simulink model "AttitudeControl_Sim"  (R2017b)
settings: Solver=ode4  StartTime=0.0  StopTime=10  FixedStep=0.001  RelTol=1e-3
InitFcn:
  | if exist('Init_control.m','file')
  | Init_control;
  | end
values from neighbouring files (symbols this model uses):
  DEG2RAD = 0.0174533    [Init_control.m]
  Kd_YAW_AngleRate = 0.00    (= 0)    [Init_control.m]
  Ki_YAW_AngleRate = 0.01    [Init_control.m]
  Kp_YAW_AngleRate = 0.5    [Init_control.m]
  MAX_CONTROL_ANGLE_PITCH = 35    [Init_control.m]
  MAX_CONTROL_ANGLE_RATE_PITCH = 220    [Init_control.m]
  MAX_CONTROL_ANGLE_RATE_ROLL = 220    [Init_control.m]
  MAX_CONTROL_ANGLE_RATE_Y = 200    [Init_control.m]
  MAX_CONTROL_ANGLE_ROLL = 35    [Init_control.m]
  ModelInit_AngEuler = [0, 0, 0]    [Init.m]    (also in Init_control.m)
  ModelInit_PosE = [0, 0, 0]    [Init.m]    (also in Init_control.m)
  ModelInit_Rads = 0    [Init.m]    (also in Init_control.m)
  ModelInit_RateB = [0, 0, 0]    [Init.m]    (also in Init_control.m)
  ModelInit_VelB = [0, 0, 0]    [Init.m]    (also in Init_control.m)
  ModelParam_envGravityAcc = 9.8    [Init.m]
  ModelParam_motorCr = 1148    [Init.m]
  ModelParam_motorJm = 0.0001287    [Init.m]
  ModelParam_motorT = 0.02    [Init.m]
  ModelParam_motorWb = -141.4    [Init.m]
  ModelParam_rotorCm = 1.779e-07    [Init.m]
  ModelParam_rotorCt = 1.105e-05    [Init.m]
  ModelParam_uavCCm = [0.0035 0.0039 0.0034]    [Init.m]
  ModelParam_uavCd = 0.055    [Init.m]
  ModelParam_uavJ = [ModelParam_uavJxx, 0, 0;     0, ModelParam_uavJyy, 0;     0, 0, ModelParam_uavJzz]    [Init.m]
  ModelParam_uavMass = 1.4    [Init.m]
  ModelParam_uavR = 0.225    [Init.m]
  Saturation_I_Y_Max = 0.2    [Init_control.m]
  Saturation_I_Y_Min = -0.2    [Init_control.m]
  THR_HOVER = 0.609    [Init_control.m]
undefined symbols (not defined in the file or in its folder): DiscIntNeverNeededParam
libraries: simulink x2, sharedutil x2, etargetslib x2, dspnetwork x1
settings Model: Creator=wsh  LastModifiedBy=张佳明
settings DebuggingCC: BusObjectLabelMismatch=error
settings CodeAppCC: StateflowObjectComments=on

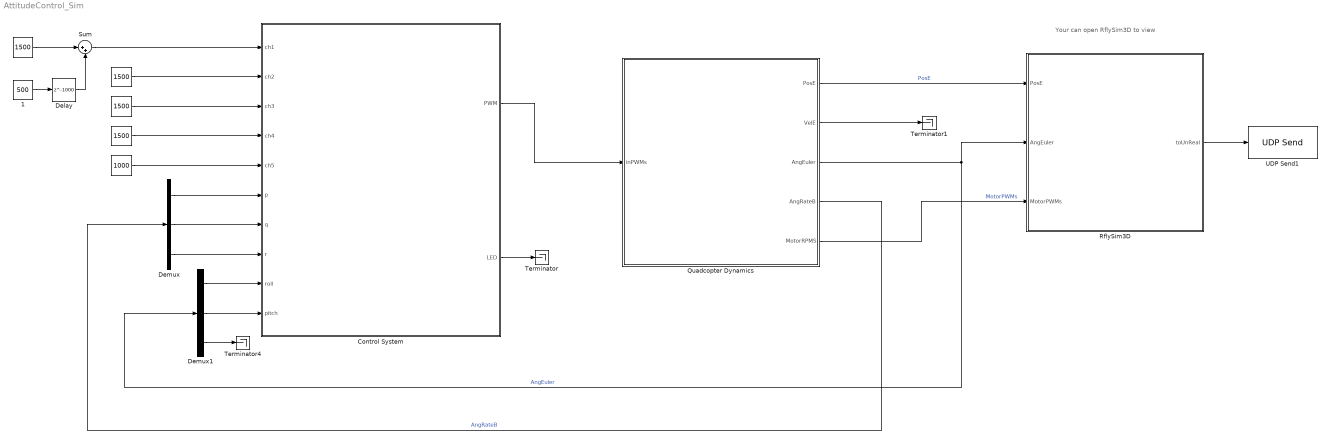
== system AttitudeControl_Sim ==
  note: Your can open RflySim3D to view
  " " : Constant  Value=1000  OutDataTypeStr=uint16
  "  " : Constant  Value=1500  OutDataTypeStr=uint16
  "   " : Constant  Value=1500  OutDataTypeStr=uint16
  "      " : Constant  Value=1500  OutDataTypeStr=uint16
  "          " : Constant  Value=1500  OutDataTypeStr=uint16
  "  1" : Constant  Value=500  OutDataTypeStr=uint16
  Control System : Subsystem
      mask Display: image('icon\pixhawk.png');
  Delay : Delay  DelayLength=1000  InitialCondition=0  SampleTime=0.001
  Demux : Demux  Outputs=3
  Demux1 : Demux  Outputs=3
  Quadcopter Dynamics : Subsystem
      mask Display: image('./icon/F450.png');
  RflySim3D : Subsystem
      mask Display: image('./icon/UE_Logo.jpg');
  Sum : Sum  Inputs=|++
  Terminator : Terminator
  Terminator1 : Terminator
  Terminator4 : Terminator
  UDP Send1 : dspnetwork/UDP Send  remoteURL='127.0.0.1'  remotePort=20010  localURL='0.0.0.0'  localPortSource=Automatically determine  localPort=-1  sampletime=-1  blockPlatform=[]  separateLengthPort=0
      settings: SourceProductName=DSP System Toolbox  SourceProductBaseCode=DS
  wires:
  Quadcopter Dynamics/1(PosE) -> RflySim3D/1(PosE)  "PosE"
  Quadcopter Dynamics/5(MotorRPMS) -> RflySim3D/3(MotorPWMs)  "MotorPWMs"
  Control System/2(LED) -> Terminator/1
  Quadcopter Dynamics/3(AngEuler) -> RflySim3D/2(AngEuler), Demux1/1  "AngEuler"
  Quadcopter Dynamics/4(AngRateB) -> Demux/1  "AngRateB"
  Demux/1 -> Control System/6(p)
  Demux/2 -> Control System/7(q)
  Demux/3 -> Control System/8(r)
  Demux1/1 -> Control System/9(roll)
  Demux1/2 -> Control System/10(pitch)
  Demux1/3 -> Terminator4/1
  Quadcopter Dynamics/2(VelE) -> Terminator1/1
  Control System/1(PWM) -> Quadcopter Dynamics/1(inPWMs)
  Delay/1 -> Sum/2
  "  1"/1 -> Delay/1
  Sum/1 -> Control System/1(ch1)
  "  "/1 -> Sum/1
  " "/1 -> Control System/5(ch5)
  "      "/1 -> Control System/3(ch3)
  "          "/1 -> Control System/4(ch4)
  "   "/1 -> Control System/2(ch2)
  RflySim3D/1(toUnReal) -> UDP Send1/1

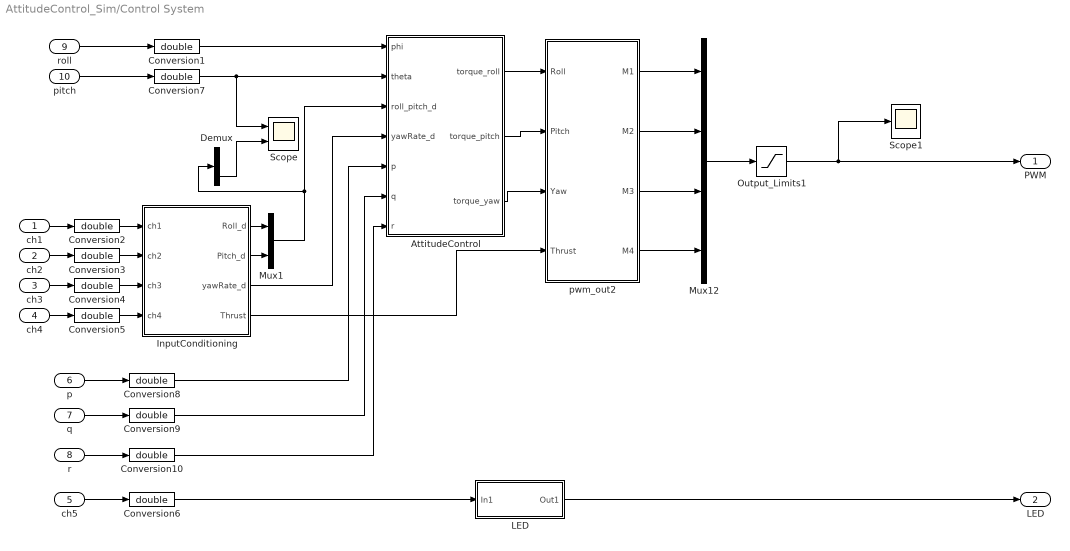
== system AttitudeControl_Sim/Control System ==
  ch1 : Inport  OutDataTypeStr=uint16  PortDimensions=1
  ch2 : Inport  Port=2  OutDataTypeStr=uint16  PortDimensions=1
  ch3 : Inport  Port=3  OutDataTypeStr=uint16  PortDimensions=1
  ch4 : Inport  Port=4  OutDataTypeStr=uint16  PortDimensions=1
  ch5 : Inport  Port=5  OutDataTypeStr=uint16  PortDimensions=1  Interpolate=off
  p : Inport  Port=6  PortDimensions=1
  q : Inport  Port=7  PortDimensions=1
  r : Inport  Port=8  PortDimensions=1
  roll : Inport  Port=9  PortDimensions=1
  pitch : Inport  Port=10  PortDimensions=1
  AttitudeControl : Subsystem
  Conversion{1..10} (10 alike) : DataTypeConversion  OutDataTypeStr=double
  Demux : Demux  Outputs=2
  InputConditioning : Subsystem
  "LED " : Subsystem
  Mux1 : Mux  Inputs=2
  Mux12 : Mux
  Output_Limits1 : Saturate  UpperLimit=2000  LowerLimit=1000
  Scope : Scope  NumInputPorts=2
  Scope1 : Scope
  pwm_out2 : MATLAB Function  SystemSampleTime=0.004
  PWM : Outport
  LED : Outport  Port=2  PortDimensions=1
  wires:
  Mux12/1 -> Output_Limits1/1
  AttitudeControl/2(torque_pitch) -> pwm_out2/2(Pitch)
  AttitudeControl/1(torque_roll) -> pwm_out2/1(Roll)
  ch3/1 -> Conversion4/1
  pwm_out2/1(M1) -> Mux12/1
  ch5/1 -> Conversion6/1
  pwm_out2/3(M3) -> Mux12/3
  pwm_out2/2(M2) -> Mux12/2
  r/1 -> Conversion10/1
  AttitudeControl/3(torque_yaw) -> pwm_out2/3(Yaw)
  Mux1/1 -> AttitudeControl/3(roll_pitch_d), Demux/1
  q/1 -> Conversion9/1
  InputConditioning/3(yawRate_d) -> AttitudeControl/4(yawRate_d)
  p/1 -> Conversion8/1
  ch4/1 -> Conversion5/1
  pwm_out2/4(M4) -> Mux12/4
  "LED "/1(Out1) -> LED/1
  Conversion6/1 -> "LED "/1(In1)
  Conversion5/1 -> InputConditioning/4(ch4)
  Conversion4/1 -> InputConditioning/3(ch3)
  pitch/1 -> Conversion7/1
  Demux/2 -> Scope/2
  roll/1 -> Conversion1/1
  Output_Limits1/1 -> PWM/1, Scope1/1
  ch1/1 -> Conversion2/1
  ch2/1 -> Conversion3/1
  InputConditioning/1(Roll_d) -> Mux1/1
  InputConditioning/2(Pitch_d) -> Mux1/2
  Conversion1/1 -> AttitudeControl/1(phi)
  Conversion7/1 -> AttitudeControl/2(theta), Scope/1
  Conversion8/1 -> AttitudeControl/5(p)
  Conversion9/1 -> AttitudeControl/6(q)
  Conversion10/1 -> AttitudeControl/7(r)
  InputConditioning/4(Thrust) -> pwm_out2/4(Thrust)
  Conversion2/1 -> InputConditioning/1("ch1 ")
  Conversion3/1 -> InputConditioning/2(ch2)

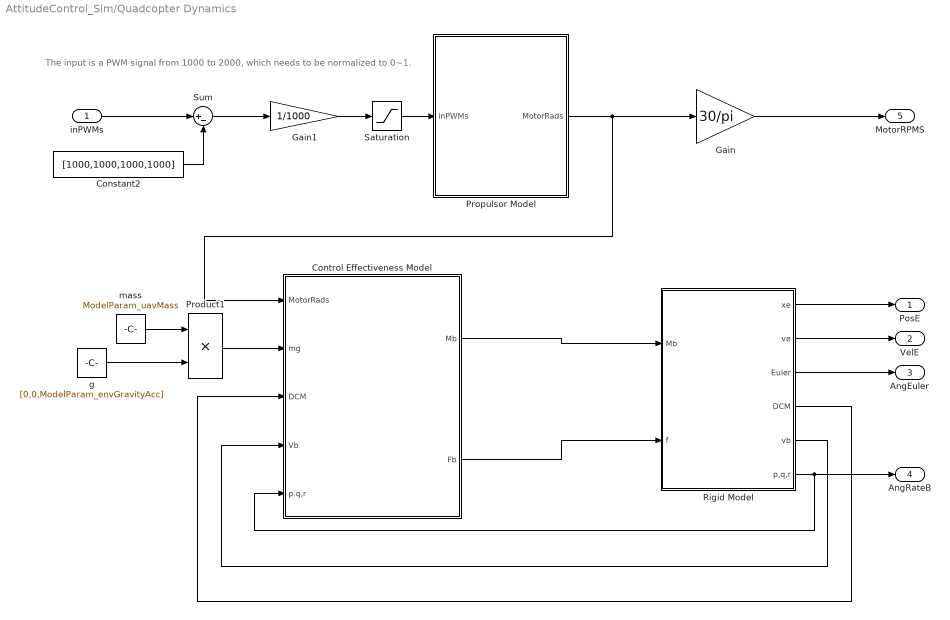
== system AttitudeControl_Sim/Quadcopter Dynamics ==
  note: The input is a PWM signal from 1000 to 2000,
      | which needs to be normalized to 0~1.
  inPWMs : Inport
  Constant2 : Constant  Value=[1000,1000,1000,1000]
  Control Effectiveness Model : Subsystem
  Gain : Gain  Gain=30/pi
  Gain1 : Gain  Gain=1/1000
  Product1 : Product
  Propulsor Model : Subsystem
  Rigid Model : Subsystem
  Saturation : Saturate  UpperLimit=1  LowerLimit=0
  Sum : Sum  Inputs=|+-
  g : Constant  Value=[0,0,ModelParam_envGravityAcc]
  mass : Constant  Value=ModelParam_uavMass
  PosE : Outport
  VelE : Outport  Port=2
  AngEuler : Outport  Port=3
  AngRateB : Outport  Port=4
  MotorRPMS : Outport  Port=5
  wires:
  Saturation/1 -> Propulsor Model/1(inPWMs)
  Rigid Model/6("p,q,r ") -> Control Effectiveness Model/5(p.q,r), AngRateB/1
  mass/1 -> Product1/1
  Rigid Model/4(DCM) -> Control Effectiveness Model/3(DCM)
  Propulsor Model/1(MotorRads) -> Gain/1, Control Effectiveness Model/1(MotorRads)
  Gain1/1 -> Saturation/1
  Rigid Model/2(ve) -> VelE/1
  Sum/1 -> Gain1/1
  Product1/1 -> Control Effectiveness Model/2(mg)
  Rigid Model/5("vb ") -> Control Effectiveness Model/4(Vb)
  Rigid Model/1("xe ") -> PosE/1
  Rigid Model/3(Euler) -> AngEuler/1
  Control Effectiveness Model/1(Mb) -> Rigid Model/1(Mb)
  inPWMs/1 -> Sum/1
  Control Effectiveness Model/2(Fb) -> Rigid Model/2(f)
  Constant2/1 -> Sum/2
  g/1 -> Product1/2
  Gain/1 -> MotorRPMS/1

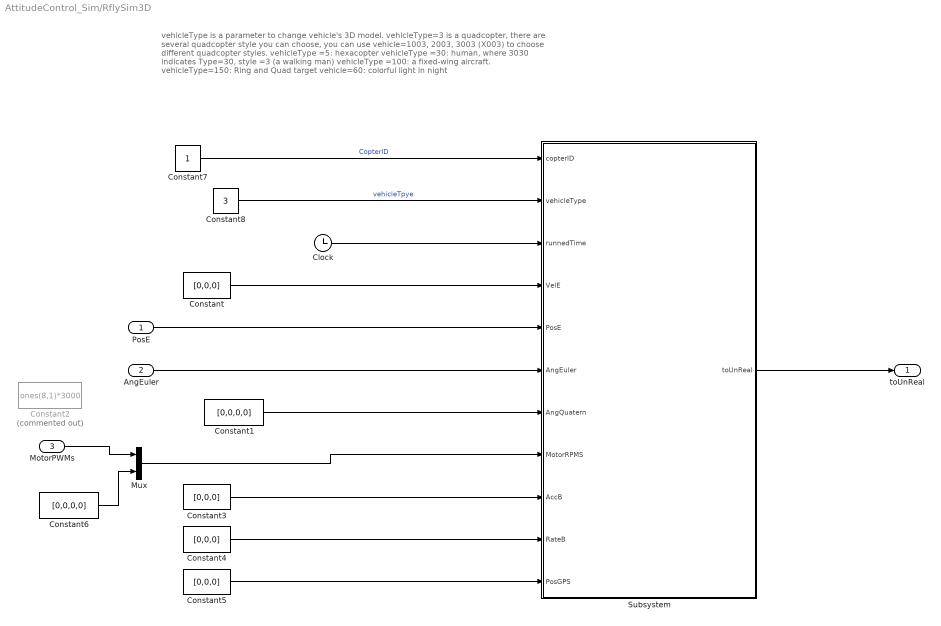
== system AttitudeControl_Sim/RflySim3D ==
  note: vehicleType is a parameter to change vehicle's 3D model.
      | vehicleType=3 is a quadcopter, there are several quadcopter style you can choose, you can use vehicle=1003, 2003, 3003 (X003) to choose different quadcopter styles.
      | vehicleType =5: hexacopter
      | vehicleType =30: human, where 3030 indicates Type=30, style =3 (a walking man)
      | vehicleType =100: a fixed-wing aircraft.
      | vehicleType=150: Ring and Quad target
      | vehicle=60: colorful light in night
  PosE : Inport  PortDimensions=3
  AngEuler : Inport  Port=2  PortDimensions=3
  MotorPWMs : Inport  Port=3  PortDimensions=4
  Clock : Clock
  Constant{,3..5} (4 alike) : Constant  Value=[0,0,0]
  Constant1 : Constant  Value=[0,0,0,0]
  Constant2 : Constant  Commented=on  Value=ones(8,1)*3000
  Constant6 : Constant  Value=[0,0,0,0]
  Constant7 : Constant
  Constant8 : Constant  Value=3
  Mux : Mux  Inputs=2
  Subsystem : Subsystem
  toUnReal : Outport
  wires:
  Constant/1 -> Subsystem/4("VelE ")
  PosE/1 -> Subsystem/5(PosE)
  Clock/1 -> Subsystem/3(runnedTime)
  Constant4/1 -> Subsystem/10(RateB)
  Constant5/1 -> Subsystem/11(PosGPS)
  AngEuler/1 -> Subsystem/6(AngEuler)
  Subsystem/1(toUnReal) -> toUnReal/1
  Constant3/1 -> Subsystem/9(AccB)
  Constant1/1 -> Subsystem/7(AngQuatern)
  Mux/1 -> Subsystem/8(MotorRPMS)
  Constant6/1 -> Mux/2
  MotorPWMs/1 -> Mux/1
  Constant7/1 -> Subsystem/1(copterID)  "CopterID"
  Constant8/1 -> Subsystem/2(vehicleType)  "vehicleTpye"

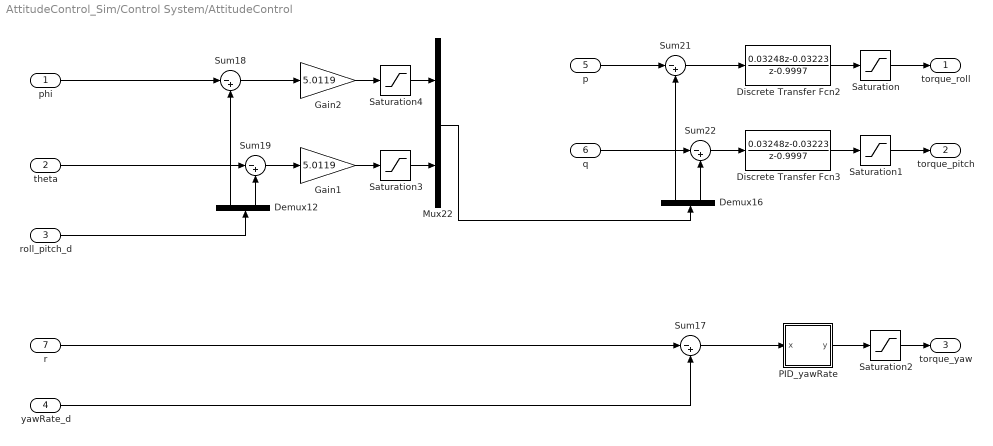
== system AttitudeControl_Sim/Control System/AttitudeControl ==
  phi : Inport
  theta : Inport  Port=2
  roll_pitch_d : Inport  Port=3
  yawRate_d : Inport  Port=4
  p : Inport  Port=5
  q : Inport  Port=6
  r : Inport  Port=7
  Demux12 : Demux  Outputs=2
  Demux16 : Demux  Outputs=2
  Discrete Transfer Fcn2 : DiscreteTransferFcn  Numerator=[0.03248 -0.03223]  Denominator=[1 -0.9997]
  Discrete Transfer Fcn3 : DiscreteTransferFcn  Numerator=[0.03248 -0.03223]  Denominator=[1 -0.9997]
  Gain1 : Gain  Gain=5.0119
  Gain2 : Gain  Gain=5.0119
  Mux22 : Mux  Inputs=2
  PID_yawRate : Subsystem
  Saturation : Saturate  UpperLimit=1  LowerLimit=-1
  Saturation1 : Saturate  UpperLimit=1  LowerLimit=-1
  Saturation2 : Saturate
  Saturation3 : Saturate  UpperLimit=MAX_CONTROL_ANGLE_RATE_PITCH  LowerLimit=-MAX_CONTROL_ANGLE_RATE_PITCH
  Saturation4 : Saturate  UpperLimit=MAX_CONTROL_ANGLE_RATE_ROLL  LowerLimit=-MAX_CONTROL_ANGLE_RATE_ROLL
  Sum{17..19,21..22} (5 alike) : Sum  Inputs=|-+
  torque_roll : Outport
  torque_pitch : Outport  Port=2
  torque_yaw : Outport  Port=3
  wires:
  r/1 -> Sum17/1
  Sum19/1 -> Gain1/1
  Gain1/1 -> Saturation3/1
  Gain2/1 -> Saturation4/1
  roll_pitch_d/1 -> Demux12/1
  Demux12/1 -> Sum18/2
  Demux12/2 -> Sum19/2
  phi/1 -> Sum18/1
  theta/1 -> Sum19/1
  Sum18/1 -> Gain2/1
  Sum22/1 -> Discrete Transfer Fcn3/1
  Sum17/1 -> PID_yawRate/1(x)
  p/1 -> Sum21/1
  q/1 -> Sum22/1
  Sum21/1 -> Discrete Transfer Fcn2/1
  Demux16/1 -> Sum21/2
  Discrete Transfer Fcn3/1 -> Saturation1/1
  Discrete Transfer Fcn2/1 -> Saturation/1
  PID_yawRate/1(y) -> Saturation2/1
  yawRate_d/1 -> Sum17/2
  Saturation/1 -> torque_roll/1
  Saturation1/1 -> torque_pitch/1
  Saturation2/1 -> torque_yaw/1
  Mux22/1 -> Demux16/1
  Saturation4/1 -> Mux22/1
  Saturation3/1 -> Mux22/2
  Demux16/2 -> Sum22/2

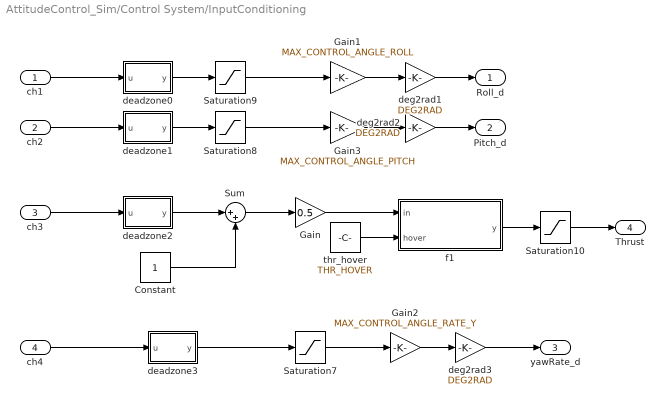
== system AttitudeControl_Sim/Control System/InputConditioning ==
  "ch1 " : Inport
  ch2 : Inport  Port=2
  ch3 : Inport  Port=3
  ch4 : Inport  Port=4
  Constant : Constant
  Gain : Gain  Gain=0.5
  Gain1 : Gain  Gain=MAX_CONTROL_ANGLE_ROLL  OutDataTypeStr=Inherit: Inherit via back propagation
  Gain2 : Gain  Gain=MAX_CONTROL_ANGLE_RATE_Y
  Gain3 : Gain  Gain=MAX_CONTROL_ANGLE_PITCH  OutDataTypeStr=Inherit: Inherit via back propagation
  Saturation10 : Saturate  UpperLimit=1  LowerLimit=0
  Saturation7 : Saturate  UpperLimit=1  LowerLimit=-1
  Saturation8 : Saturate  UpperLimit=1  LowerLimit=-1
  Saturation9 : Saturate  UpperLimit=1  LowerLimit=-1
  Sum : Sum  Inputs=|++
  deadzone0 : MATLAB Function  TreatAsAtomicUnit=on
  deadzone1 : MATLAB Function  TreatAsAtomicUnit=on
  deadzone2 : MATLAB Function  TreatAsAtomicUnit=on
  deadzone3 : MATLAB Function  TreatAsAtomicUnit=on
  deg2rad1 : Gain  Gain=DEG2RAD
  deg2rad2 : Gain  Gain=DEG2RAD
  deg2rad3 : Gain  Gain=DEG2RAD
  f1 : MATLAB Function  TreatAsAtomicUnit=on
  "thr_hover " : Constant  Value=THR_HOVER
  Roll_d : Outport
  Pitch_d : Outport  Port=2
  yawRate_d : Outport  Port=3
  Thrust : Outport  Port=4
  wires:
  deadzone2/1(y) -> Sum/1
  ch3/1 -> deadzone2/1(u)
  deadzone1/1(y) -> Saturation8/1
  Saturation10/1 -> Thrust/1
  deadzone0/1(y) -> Saturation9/1
  "ch1 "/1 -> deadzone0/1(u)
  ch2/1 -> deadzone1/1(u)
  Saturation9/1 -> Gain1/1
  Saturation8/1 -> Gain3/1
  Gain3/1 -> deg2rad2/1
  Constant/1 -> Sum/2
  Sum/1 -> Gain/1
  Gain1/1 -> deg2rad1/1
  deg2rad1/1 -> Roll_d/1
  deg2rad2/1 -> Pitch_d/1
  Saturation7/1 -> Gain2/1
  deadzone3/1(y) -> Saturation7/1
  ch4/1 -> deadzone3/1(u)
  Gain2/1 -> deg2rad3/1
  deg2rad3/1 -> yawRate_d/1
  "thr_hover "/1 -> f1/2(hover)
  Gain/1 -> f1/1(in)
  f1/1(y) -> Saturation10/1

== system AttitudeControl_Sim/Control System/LED  ==
  In1 : Inport
  Compare To Constant3 : simulink/Logic and Bit Operations/Compare To Constant  relop=>=  const=uint16(1500)  OutDataTypeStr=boolean
  Out1 : Outport
  wires:
  Compare To Constant3/1 -> Out1/1
  In1/1 -> Compare To Constant3/1

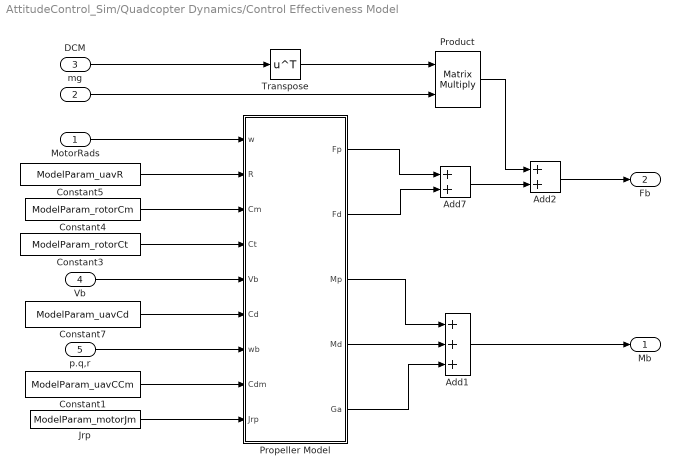
== system AttitudeControl_Sim/Quadcopter Dynamics/Control Effectiveness Model ==
  MotorRads : Inport
  mg : Inport  Port=2
  DCM : Inport  Port=3
  Vb : Inport  Port=4
  p.q,r : Inport  Port=5
  Add1 : Sum  Inputs=+++
  Add2 : Sum
  Add7 : Sum
  Constant1 : Constant  Value=ModelParam_uavCCm
  Constant3 : Constant  Value=ModelParam_rotorCt
  Constant4 : Constant  Value=ModelParam_rotorCm
  Constant5 : Constant  Value=ModelParam_uavR
  Constant7 : Constant  Value=ModelParam_uavCd
  Jrp : Constant  Value=ModelParam_motorJm
  Product : Product  Multiplication=Matrix(*)
  Propeller Model : MATLAB Function  TreatAsAtomicUnit=on
  Transpose : Math  Operator=transpose  SaturateOnIntegerOverflow=on
  Mb : Outport
  Fb : Outport  Port=2
  wires:
  Add2/1 -> Fb/1
  Constant3/1 -> Propeller Model/4(Ct)
  Propeller Model/2(Fd) -> Add7/2
  Add7/1 -> Add2/2
  Propeller Model/1(Fp) -> Add7/1
  Product/1 -> Add2/1
  mg/1 -> Product/2
  DCM/1 -> Transpose/1
  Constant7/1 -> Propeller Model/6(Cd)
  Vb/1 -> Propeller Model/5(Vb)
  Constant5/1 -> Propeller Model/2(R)
  Constant4/1 -> Propeller Model/3(Cm)
  MotorRads/1 -> Propeller Model/1(w)
  Transpose/1 -> Product/1
  Propeller Model/3(Mp) -> Add1/1
  Propeller Model/4(Md) -> Add1/2
  Add1/1 -> Mb/1
  p.q,r/1 -> Propeller Model/7(wb)
  Constant1/1 -> Propeller Model/8(Cdm)
  Jrp/1 -> Propeller Model/9(Jrp)
  Propeller Model/5(Ga) -> Add1/3

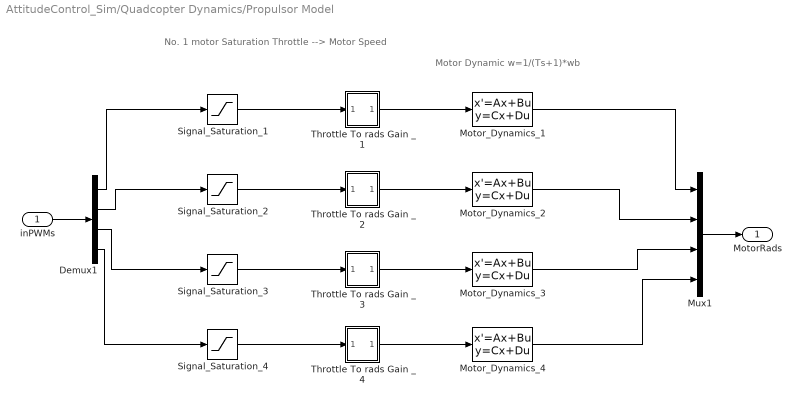
== system AttitudeControl_Sim/Quadcopter Dynamics/Propulsor Model ==
  note: Motor Dynamic
      | w=1/(Ts+1)*wb
  note: No. 1 motor
      |
      |          Saturation             Throttle --> Motor Speed
  inPWMs : Inport
  Demux1 : Demux
  Motor_Dynamics_{1..4} (4 alike) : StateSpace  A=-1/ModelParam_motorT  C=1/ModelParam_motorT  D=0  InitialCondition=ModelInit_Rads*ModelParam_motorT
  Mux1 : Mux
  Signal_Saturation_{1..4} (4 alike) : Saturate  UpperLimit=1  LowerLimit=0
  Throttle To rads Gain _1 : Subsystem
  Throttle To rads Gain _2 : Subsystem
  Throttle To rads Gain _3 : Subsystem
  Throttle To rads Gain _4 : Subsystem
  MotorRads : Outport
  wires:
  Throttle To rads Gain _4/1(Out5) -> Motor_Dynamics_4/1
  Signal_Saturation_4/1 -> Throttle To rads Gain _4/1(In5)
  Signal_Saturation_3/1 -> Throttle To rads Gain _3/1(In5)
  Signal_Saturation_2/1 -> Throttle To rads Gain _2/1(In5)
  Motor_Dynamics_4/1 -> Mux1/4
  Motor_Dynamics_3/1 -> Mux1/3
  Motor_Dynamics_2/1 -> Mux1/2
  Motor_Dynamics_1/1 -> Mux1/1
  Signal_Saturation_1/1 -> Throttle To rads Gain _1/1(In5)
  Mux1/1 -> MotorRads/1
  Throttle To rads Gain _3/1(Out5) -> Motor_Dynamics_3/1
  Throttle To rads Gain _2/1(Out5) -> Motor_Dynamics_2/1
  Throttle To rads Gain _1/1(Out5) -> Motor_Dynamics_1/1
  inPWMs/1 -> Demux1/1
  Demux1/4 -> Signal_Saturation_4/1
  Demux1/3 -> Signal_Saturation_3/1
  Demux1/2 -> Signal_Saturation_2/1
  Demux1/1 -> Signal_Saturation_1/1

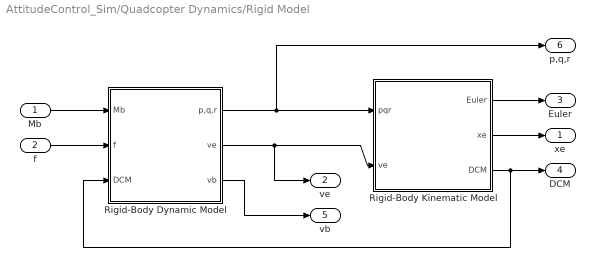
== system AttitudeControl_Sim/Quadcopter Dynamics/Rigid Model ==
  Mb : Inport
  f : Inport  Port=2
  Rigid-Body Dynamic Model : Subsystem
  "Rigid-Body Kinematic Model " : Subsystem
  "xe " : Outport
  ve : Outport  Port=2
  Euler : Outport  Port=3
  DCM : Outport  Port=4
  "vb " : Outport  Port=5
  "p,q,r " : Outport  Port=6
  wires:
  Rigid-Body Dynamic Model/1("p,q,r ") -> "Rigid-Body Kinematic Model "/1(pqr), "p,q,r "/1
  "Rigid-Body Kinematic Model "/1(Euler) -> Euler/1
  "Rigid-Body Kinematic Model "/3(DCM) -> Rigid-Body Dynamic Model/3(DCM), DCM/1
  Mb/1 -> Rigid-Body Dynamic Model/1(Mb)
  f/1 -> Rigid-Body Dynamic Model/2(f)
  Rigid-Body Dynamic Model/2(ve) -> "Rigid-Body Kinematic Model "/2(ve), ve/1
  Rigid-Body Dynamic Model/3("vb ") -> "vb "/1
  "Rigid-Body Kinematic Model "/2("xe ") -> "xe "/1

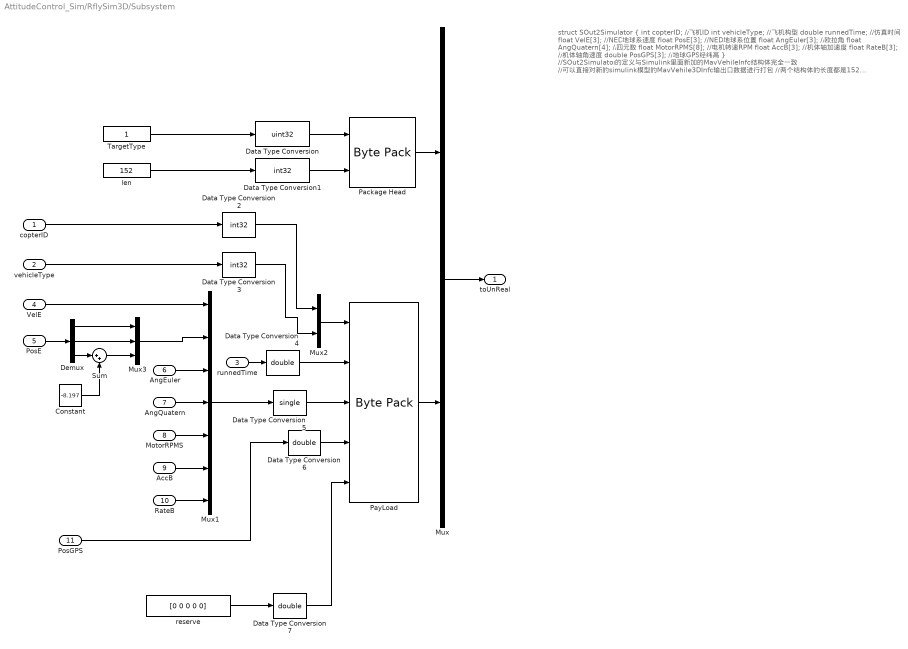
== system AttitudeControl_Sim/RflySim3D/Subsystem ==
  note: struct SOut2Simulator
      | {
      | int copterID; //飞机ID
      | int vehicleType; //飞机构型
      | double runnedTime; //仿真时间
      | float VelE[3]; //NED地球系速度
      | float PosE[3]; //NED地球系位置
      | float AngEuler[3]; //欧拉角
      | float AngQuatern[4]; //四元数
      | float MotorRPMS[8]; //电机转速RPM
      | float AccB[3]; //机体轴加速度
      | float RateB[3]; //机体轴角速度
      | double PosGPS[3]; //地球GPS经纬高
      | }
      |
      | //SOut2Simulator的定义与Simulink里面新加的MavVehileInfo结构体完全一致
      | //可以直接对新的simulink模型的MavVehile3DInfo输出口数据进行打包
      | //两个结构体的长度都是152
      | sizeof(SOut2Simulator) = sizeof(MavVehileInfo) = 152
      |
      | 打包封装的结构体为
      | typedef struct _netDataShort
      | {
      | TargetType tg; //这里目前随便填，写1即可 uint32
      | int len; //这个长度为传输结构体长度，目前是152
      | char payload[192]; //这里面前152位存放了SOut2Simulator结构体数据，后面的40位保留
      | }netDataShort;
      |
      | //UDP包的总长度为200
      | sizeof(netDataShort) = 200
      |
      | //发送的UDP端口号为：20010
  copterID : Inport  PortDimensions=1
  vehicleType : Inport  Port=2  PortDimensions=1
  runnedTime : Inport  Port=3  PortDimensions=1
  "VelE " : Inport  Port=4  PortDimensions=3
  PosE : Inport  Port=5  PortDimensions=3
  AngEuler : Inport  Port=6  PortDimensions=3
  AngQuatern : Inport  Port=7  PortDimensions=4
  MotorRPMS : Inport  Port=8  PortDimensions=8
  AccB : Inport  Port=9  PortDimensions=3
  RateB : Inport  Port=10  PortDimensions=3
  PosGPS : Inport  Port=11  PortDimensions=3
  Constant : Constant  Value=-8.197
  Data Type Conversion : DataTypeConversion  OutDataTypeStr=uint32
  Data Type Conversion1 : DataTypeConversion  OutDataTypeStr=int32
  Data Type Conversion2 : DataTypeConversion  OutDataTypeStr=int32
  Data Type Conversion3 : DataTypeConversion  OutDataTypeStr=int32
  Data Type Conversion4 : DataTypeConversion  OutDataTypeStr=double
  Data Type Conversion5 : DataTypeConversion  OutDataTypeStr=single
  Data Type Conversion6 : DataTypeConversion  OutDataTypeStr=double
  Data Type Conversion7 : DataTypeConversion  OutDataTypeStr=double
  Demux : Demux  Outputs=3
  Mux : Mux  Inputs=2
  Mux1 : Mux  Inputs=7
  Mux2 : Mux  Inputs=2
  Mux3 : Mux  Inputs=3
  Package Head : etargetslib/Byte Pack  datatypes={'uint32','int32'}  byteAlign=4
      settings: SourceProductName=MATLAB Coder
  PayLoad : etargetslib/Byte Pack  datatypes={'int32','double','single','double','double'}  byteAlign=8
      settings: SourceProductName=MATLAB Coder
  Sum : Sum  Inputs=|++
  TargetType : Constant  OutDataTypeStr=Inherit: Inherit via back propagation
  len : Constant  Value=152  OutDataTypeStr=Inherit: Inherit via back propagation
  reserve : Constant  Value=[0 0 0 0 0]  OutDataTypeStr=double
  toUnReal : Outport
  wires:
  runnedTime/1 -> Data Type Conversion4/1
  RateB/1 -> Mux1/7
  PayLoad/1 -> Mux/2
  "VelE "/1 -> Mux1/1
  Mux1/1 -> Data Type Conversion5/1
  PosGPS/1 -> Data Type Conversion6/1
  Package Head/1 -> Mux/1
  AccB/1 -> Mux1/6
  Mux/1 -> toUnReal/1
  MotorRPMS/1 -> Mux1/5
  AngQuatern/1 -> Mux1/4
  copterID/1 -> Data Type Conversion2/1
  len/1 -> Data Type Conversion1/1
  vehicleType/1 -> Data Type Conversion3/1
  TargetType/1 -> Data Type Conversion/1
  reserve/1 -> Data Type Conversion7/1
  Mux2/1 -> PayLoad/1
  AngEuler/1 -> Mux1/3
  Data Type Conversion5/1 -> PayLoad/3
  Data Type Conversion2/1 -> Mux2/1
  Data Type Conversion1/1 -> Package Head/2
  Data Type Conversion6/1 -> PayLoad/4
  Data Type Conversion/1 -> Package Head/1
  Data Type Conversion3/1 -> Mux2/2
  Data Type Conversion4/1 -> PayLoad/2
  Data Type Conversion7/1 -> PayLoad/5
  PosE/1 -> Demux/1
  Demux/3 -> Sum/1
  Sum/1 -> Mux3/3
  Constant/1 -> Sum/2
  Demux/1 -> Mux3/1
  Demux/2 -> Mux3/2
  Mux3/1 -> Mux1/2

== system AttitudeControl_Sim/Control System/AttitudeControl/PID_yawRate ==
  x : Inport
  Derivative Gain : Gain  DisableCoverage=on  Gain=Kd_YAW_AngleRate  ParamMin=-100  ParamMax=100  OutMin=-100  OutMax=100
  Discrete Derivative : simulink/Discrete/Discrete Derivative  gainval=1.0  ICPrevScaledInput=0.0  OutMin=[]  OutMax=[]  OutDataType=fixdt(1, 16)  OutScaling=2^-10  DoSatur=off
  Discrete-Time Integrator : DiscreteIntegrator  InitialConditionSetting=State (most efficient)  SampleTime=-1  LimitOutput=on  UpperSaturationLimit=Saturation_I_Y_Max  LowerSaturationLimit=Saturation_I_Y_Min  ICPrevOutput=DiscIntNeverNeededParam  ICPrevScaledInput=DiscIntNeverNeededParam
  Gain : Gain  Gain=Kp_YAW_AngleRate
  Integral Gain : Gain  DisableCoverage=on  Gain=Ki_YAW_AngleRate
  Sum : Sum  Inputs=+++
  y : Outport  InitialOutput=0
  wires:
  x/1 -> Gain/1, Integral Gain/1, Derivative Gain/1
  Integral Gain/1 -> Discrete-Time Integrator/1
  Derivative Gain/1 -> Discrete Derivative/1
  Gain/1 -> Sum/1
  Sum/1 -> y/1
  Discrete Derivative/1 -> Sum/3
  Discrete-Time Integrator/1 -> Sum/2

== system AttitudeControl_Sim/Quadcopter Dynamics/Propulsor Model/Throttle To rads Gain _1 ==
  In5 : Inport
  Constant : Constant  Value=ModelParam_motorWb
  Gain : Gain  Gain=ModelParam_motorCr
  Sum1 : Sum  Inputs=++|
  Out5 : Outport
  wires:
  Constant/1 -> Sum1/1
  Gain/1 -> Sum1/2
  In5/1 -> Gain/1
  Sum1/1 -> Out5/1

== system AttitudeControl_Sim/Quadcopter Dynamics/Propulsor Model/Throttle To rads Gain _2 ==
  In5 : Inport
  Constant : Constant  Value=ModelParam_motorWb
  Gain : Gain  Gain=ModelParam_motorCr
  Sum1 : Sum  Inputs=++|
  Out5 : Outport
  wires:
  Sum1/1 -> Out5/1
  In5/1 -> Gain/1
  Gain/1 -> Sum1/2
  Constant/1 -> Sum1/1

== system AttitudeControl_Sim/Quadcopter Dynamics/Propulsor Model/Throttle To rads Gain _3 ==
  In5 : Inport
  Constant : Constant  Value=ModelParam_motorWb
  Gain : Gain  Gain=ModelParam_motorCr
  Sum1 : Sum  Inputs=++|
  Out5 : Outport
  wires:
  Constant/1 -> Sum1/1
  Gain/1 -> Sum1/2
  In5/1 -> Gain/1
  Sum1/1 -> Out5/1

== system AttitudeControl_Sim/Quadcopter Dynamics/Propulsor Model/Throttle To rads Gain _4 ==
  In5 : Inport
  Constant : Constant  Value=ModelParam_motorWb
  Gain : Gain  Gain=ModelParam_motorCr
  Sum1 : Sum  Inputs=++|
  Out5 : Outport
  wires:
  Sum1/1 -> Out5/1
  In5/1 -> Gain/1
  Gain/1 -> Sum1/2
  Constant/1 -> Sum1/1

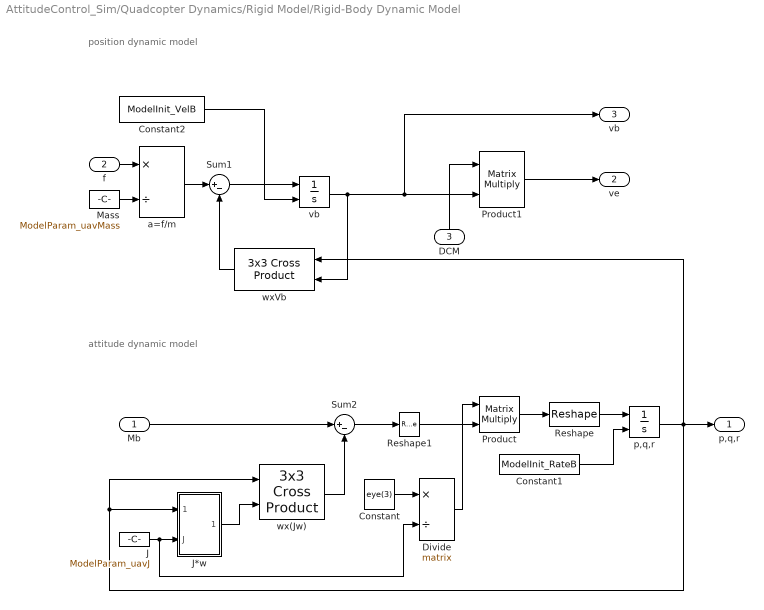
== system AttitudeControl_Sim/Quadcopter Dynamics/Rigid Model/Rigid-Body Dynamic Model ==
  note: attitude dynamic model
  note: position dynamic model
  Mb : Inport
  f : Inport  Port=2
  DCM : Inport  Port=3
  " Mass " : Constant  Value=ModelParam_uavMass
  Constant : Constant  Value=eye(3)
  Constant1 : Constant  Value=ModelInit_RateB
  Constant2 : Constant  Value=ModelInit_VelB
  Divide : Product  Inputs=*/  Multiplication=Matrix(*)
  "J " : Constant  Value=ModelParam_uavJ
  J*w : Subsystem
  Product : Product  Multiplication=Matrix(*)
  Product1 : Product  Multiplication=Matrix(*)
  Reshape : Reshape  OutputDimensionality=Customize  OutputDimensions=[3,1]
  Reshape1 : Reshape  OutputDimensionality=Column vector (2-D)
  Sum1 : Sum  Inputs=|+-
  Sum2 : Sum  Inputs=|+-
  a=f/m : Product  Inputs=*/
  p,q,r : Integrator  InitialConditionSource=external
  vb : Integrator  InitialConditionSource=external
  wx(Jw) : sharedutil/3x3 Cross Product
      settings: SourceProductBaseCode=AE
  wxVb : sharedutil/3x3 Cross Product
      settings: SourceProductBaseCode=AE
  "p,q,r " : Outport
  ve : Outport  Port=2
  "vb " : Outport  Port=3
  wires:
  Product/1 -> Reshape/1
  Reshape1/1 -> Product/2
  Constant/1 -> Divide/1
  Divide/1 -> Product/1
  Sum2/1 -> Reshape1/1
  "J "/1 -> Divide/2, J*w/2(J)
  p,q,r/1 -> "p,q,r "/1, J*w/1(p q r), wx(Jw)/1, wxVb/1
  J*w/1("J*w ") -> wx(Jw)/2
  Mb/1 -> Sum2/1
  wx(Jw)/1 -> Sum2/2
  Constant2/1 -> vb/2
  f/1 -> a=f/m/1
  Product1/1 -> ve/1
  wxVb/1 -> Sum1/2
  a=f/m/1 -> Sum1/1
  Sum1/1 -> vb/1
  vb/1 -> Product1/2, "vb "/1, wxVb/2
  " Mass "/1 -> a=f/m/2
  DCM/1 -> Product1/1
  Reshape/1 -> p,q,r/1
  Constant1/1 -> p,q,r/2

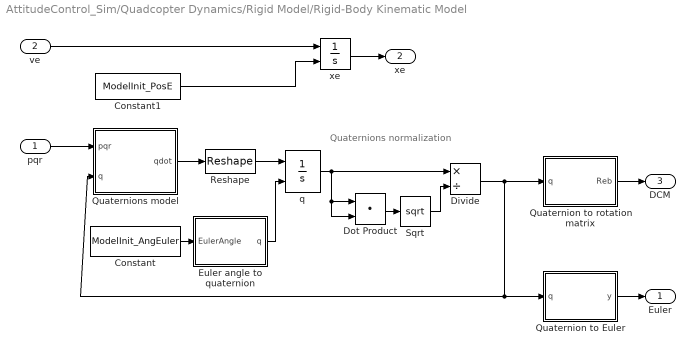
== system AttitudeControl_Sim/Quadcopter Dynamics/Rigid Model/Rigid-Body Kinematic Model  ==
  note: Quaternions
      | normalization
  pqr : Inport
  ve : Inport  Port=2
  Constant : Constant  Value=ModelInit_AngEuler
  Constant1 : Constant  Value=ModelInit_PosE
  Divide : Product  Inputs=*/
  Dot Product : DotProduct  InputSameDT=on  OutDataTypeStr=Inherit: Inherit via internal rule
  Euler angle to quaternion : MATLAB Function
  Quaternion to Euler : MATLAB Function
  Quaternion to rotation matrix : MATLAB Function
  Quaternions model : MATLAB Function  TreatAsAtomicUnit=on
  Reshape : Reshape  OutputDimensionality=Customize  OutputDimensions=[4,1]
  Sqrt : Sqrt  SaturateOnIntegerOverflow=on
  q : Integrator  InitialConditionSource=external
  xe : Integrator  InitialConditionSource=external
  Euler : Outport
  "xe " : Outport  Port=2
  DCM : Outport  Port=3
  wires:
  Divide/1 -> Quaternion to rotation matrix/1(q), Quaternions model/2(q), Quaternion to Euler/1(q)
  Dot Product/1 -> Sqrt/1
  pqr/1 -> Quaternions model/1(pqr)
  q/1 -> Divide/1, Dot Product/1, Dot Product/2
  Quaternions model/1(qdot) -> Reshape/1
  Quaternion to rotation matrix/1(Reb) -> DCM/1
  Quaternion to Euler/1(y) -> Euler/1
  Constant/1 -> Euler angle to quaternion/1(EulerAngle)
  Euler angle to quaternion/1(q) -> q/2
  Reshape/1 -> q/1
  ve/1 -> xe/1
  xe/1 -> "xe "/1
  Constant1/1 -> xe/2
  Sqrt/1 -> Divide/2

== system AttitudeControl_Sim/Quadcopter Dynamics/Rigid Model/Rigid-Body Dynamic Model/J*w ==
  p q r : Inport
  J : Inport  Port=2
  J*w : Product  Multiplication=Matrix(*)
  "J*w " : Outport
  wires:
  J*w/1 -> "J*w "/1
  J/1 -> J*w/1
  p q r/1 -> J*w/2

== matlab function AttitudeControl_Sim/Control System/InputConditioning/deadzone0 ==
  data: u input; y output
function y = fcn(u)
%Function description:
%  Control the range of the remote control input from RCMin to RCMax, and set
%  a dead zone with a dead zone size of ±deadZone,the output y is
%  normalized to 0~1.You can get the RC calibration parameters in QGC.
RCMin = 1100;
RCMax = 1900;
RCMid = (RCMin + RCMax)/2;
deadZoneRate = 0.05;
deadZone = deadZoneRate*(RCMax - RCMin);
k = 1/(RCMax - RCMid - deadZone);
%Limiting
if(u < RCMin)
    u = RCMin;
elseif(u > RCMax)
    u = RCMax;
end
%dead zone and normalize
 if(u > RCMid + deadZone)
    y = (u-RCMid - deadZone)*k;
 elseif(u < RCMid - deadZone)
     y = (u - RCMid + deadZone)*k;
 else
     y = 0;
 end

 end

== matlab function AttitudeControl_Sim/Control System/InputConditioning/deadzone1 ==
  data: u input; y output
function y = fcn(u)
%Function description:
%  Control the range of the remote control input from RCMin to RCMax, and set
%  a dead zone with a dead zone size of ±deadZone,the output y is
%  normalized to 0~1.You can get the RC calibration parameters in QGC.
RCMin = 1100;
RCMax = 1900;
RCMid = (RCMin + RCMax)/2;
deadZoneRate = 0.05;
deadZone = deadZoneRate*(RCMax - RCMin);
k = 1/(RCMax - RCMid - deadZone);
%Limiting
if(u < RCMin)
    u = RCMin;
elseif(u > RCMax)
    u = RCMax;
end
%dead zone and normalize
 if(u > RCMid + deadZone)
    y = (u-RCMid - deadZone)*k;
 elseif(u < RCMid - deadZone)
     y = (u - RCMid + deadZone)*k;
 else
     y = 0;
 end

 end

== matlab function AttitudeControl_Sim/Control System/InputConditioning/deadzone2 ==
  data: u input; y output
function y = fcn(u)
%Function description:
%  Control the range of the remote control input from RCMin to RCMax, and set
%  a dead zone with a dead zone size of ±deadZone,the output y is
%  normalized to 0~1.You can get the RC calibration parameters in QGC.
RCMin = 1100;
RCMax = 1900;
RCMid = (RCMin + RCMax)/2;
deadZoneRate = 0.05;
deadZone = deadZoneRate*(RCMax - RCMin);
k = 1/(RCMax - RCMid - deadZone);
%Limiting
if(u < RCMin)
    u = RCMin;
elseif(u > RCMax)
    u = RCMax;
end
%dead zone and normalize
 if(u > RCMid + deadZone)
    y = (u-RCMid - deadZone)*k;
 elseif(u < RCMid - deadZone)
     y = (u - RCMid + deadZone)*k;
 else
     y = 0;
 end

 end

== matlab function AttitudeControl_Sim/Control System/InputConditioning/deadzone3 ==
  data: u input; y output
function y = fcn(u)
%Function description:
%  Control the range of the remote control input from RCMin to RCMax, and set
%  a dead zone with a dead zone size of ±deadZone,the output y is
%  normalized to 0~1.You can get the RC calibration parameters in QGC.
RCMin = 1100;
RCMax = 1900;
RCMid = (RCMin + RCMax)/2;
deadZoneRate = 0.05;
deadZone = deadZoneRate*(RCMax - RCMin);
k = 1/(RCMax - RCMid - deadZone);
%Limiting
if(u < RCMin)
    u = RCMin;
elseif(u > RCMax)
    u = RCMax;
end
%dead zone and normalize
 if(u > RCMid + deadZone)
    y = (u-RCMid - deadZone)*k;
 elseif(u < RCMid - deadZone)
     y = (u - RCMid + deadZone)*k;
 else
     y = 0;
 end

 end

== matlab function AttitudeControl_Sim/Quadcopter Dynamics/Rigid Model/Rigid-Body Kinematic Model /Quaternion to rotation matrix ==
  data: q input; Reb output
function Reb = fcn(q)
%Function description;
%  The rotation matrix of the Aircraft-Body Coordinate Frame (ABCF) to the
%  Earth-Fixed Coordinate Frame (EFCF) is obtained from the quaternions
Reb = [q(1)*q(1) + q(2)*q(2) - q(3)*q(3) - q(4)*q(4), 2*(q(2)*q(3) - q(1)*q(4)), 2*(q(2)*q(4) + q(1)*q(3))
           2*(q(2)*q(3) + q(1)*q(4)), q(1)*q(1) - q(2)*q(2) + q(3)*q(3) - q(4)*q(4), 2*(q(3)*q(4) - q(1)*q(2))
           2*(q(2)*q(4) - q(1)*q(3)), 2*(q(3)*q(4) + q(1)*q(2)), q(1)*q(1) - q(2)*q(2) - q(3)*q(3) + q(4)*q(4)];

== matlab function AttitudeControl_Sim/Quadcopter Dynamics/Rigid Model/Rigid-Body Kinematic Model /Quaternion to Euler ==
  data: q input; y output
function y = fcn(q)
 %Function description:
%  Quaternions to Euler
phi = atan2(2*(q(1)*q(2) + q(3)*q(4)), (1 - 2*(q(2)*q(2) + q(3)*q(3))));
theta = asin(2*(q(1)*q(3) - q(2)*q(4)));
psi = atan2(2*(q(1)*q(4) + q(2)*q(3)), (1 - 2*(q(3)*q(3) + q(4)*q(4))));
y = [phi theta psi];

== matlab function AttitudeControl_Sim/Quadcopter Dynamics/Rigid Model/Rigid-Body Kinematic Model /Quaternions model ==
  data: pqr input; qdot output; q input
function qdot = fcn(pqr, q)
%Function description:
%  Quaternions model
qdot = 0.5*[0, -pqr(1), -pqr(2), -pqr(3); pqr(1), 0, pqr(3), -pqr(2); pqr(2), -pqr(3), 0, pqr(1); pqr(3), pqr(2), -pqr(1), 0]*q;

== matlab function AttitudeControl_Sim/Quadcopter Dynamics/Rigid Model/Rigid-Body Kinematic Model /Euler angle to quaternion ==
  data: EulerAngle input; q output
function q = fcn(EulerAngle)
%Function description:
%  Get quaternions from Euler angle
q0 =  cos(EulerAngle(1)/2)*cos(EulerAngle(2)/2)*cos(EulerAngle(3)/2) + sin(EulerAngle(1)/2)*sin((EulerAngle(2)/2))*sin((EulerAngle(3)/2));
q1 = sin(EulerAngle(1)/2)*cos(EulerAngle(2)/2)*cos(EulerAngle(3)/2) - cos(EulerAngle(1)/2)*sin((EulerAngle(2)/2))*sin((EulerAngle(3)/2));
q2 = cos(EulerAngle(1)/2)*sin(EulerAngle(2)/2)*cos(EulerAngle(3)/2) + sin(EulerAngle(1)/2)*cos((EulerAngle(2)/2))*sin((EulerAngle(3)/2));
q3 = cos(EulerAngle(1)/2)*cos(EulerAngle(2)/2)*sin(EulerAngle(3)/2) - sin(EulerAngle(1)/2)*sin((EulerAngle(2)/2))*cos((EulerAngle(3)/2));
q = [q0 q1 q2 q3]';

== matlab function AttitudeControl_Sim/Quadcopter Dynamics/Control Effectiveness Model/Propeller Model ==
  data: w input; R input; Fp output; Fd output; Mp output; Cm input; Ct input; Vb input; Cd input; wb input; Md output; Cdm input; Jrp input; Ga output
function [Fp, Fd, Mp, Md, Ga] = fcn(w, R, Cm, Ct, Vb, Cd,wb, Cdm, Jrp)
 %Function description:
 %  Obtain the force and torque acting on the body. The airframe of the
 %  quadrotor is as follows:
 %3↓   1↑
 %  \ /
 %  / \
 %2↑   4↓
 %↑ stands for counterclockwise and ↓stands for clockwise.
 %Input：
 %  w: motor speed，unit：rad/s
 %  R: body radius(m)
 %  Cm: torque coefficient
 %  Ct: thrust coefficient
 %  Vb: aircraft speed in the body coordinate system
 %  Cd: damping coefficient
 %  wb: angular velocity in the body coordinate system
 %  Cdm: damping moment coefficient vector
 %  Jrp:  moment of inertia of motor rotor + propeller
 %Output:
 %  Fp: thrust under the body coordinate system
 %  Fd: aerodynamic force under the body coordinate system
 %  Mp: torque under the body coordinate system
 %  Md: aerodynamic moment
 %  Ga: gyro moment
 M_rctcm = [-sin(pi/4)*R*Ct, sin(pi/4)*R*Ct, sin(pi/4)*R*Ct, -sin(pi/4)*R*Ct;
            sin(pi/4)*R*Ct, -sin(pi/4)*R*Ct, sin(pi/4)*R*Ct, -sin(pi/4)*R*Ct;
            Cm, Cm, -Cm, -Cm];
 Mp = M_rctcm*(w.^2);  % torque
 
 Fp = [0; 0; -sum(Ct*(w.^2))];  % thrust
 Fd = -Cd*Vb.*abs(Vb)*0.5;  % aerodynamic force
 Md = -Cdm.*wb.*abs(wb);  % aerodynamic moment
 % gyro moment
 Ga = zeros(3,1);
 Ga(1) = Jrp*wb(2)*( w(1) + w(2) - w(3) - w(4));
 Ga(2) = Jrp*wb(1)*(-w(1) - w(2) + w(3) + w(4));
end

== matlab function AttitudeControl_Sim/Control System/pwm_out2 ==
  data: Roll input; M1 output; Pitch input; Yaw input; Thrust input; M2 output; M3 output; M4 output
function [M1, M2, M3, M4] = motor_mixer(Roll, Pitch, Yaw, Thrust)
%Function description:
%  Control allocation. The quadrotor type is X-configuration,
%  and the airframe is as follows:
%3↓   1↑
 %  \ /
 %  / \
 %2↑   4↓
%Input：
%  Roll, Pitch, Yaw: attitude controller output.
%  Thrust

idle_PWM = 1000;
scale = 1000;

M1 = (Thrust - Roll + Pitch + Yaw) * scale + idle_PWM;
M2 = (Thrust + Roll - Pitch + Yaw) * scale + idle_PWM;
M3 = (Thrust + Roll + Pitch - Yaw) * scale + idle_PWM;
M4 = (Thrust - Roll - Pitch - Yaw) * scale + idle_PWM;

== matlab function AttitudeControl_Sim/Control System/InputConditioning/f1 ==
  data: in input; y output; hover input
function y = thr_curve(in, hover)
%Function description:
%  After this function, when the throttle is in the middle position, the output is hovering throttle hover
%Input:
%  in: Throttle normalized value, range (0~1)
%  hover: Hovering throttle value
%Output:
%  Processed throttle value
if in < 0.5
	y=2 * in * hover;
else
	y=hover + 2 * (in - 0.5) * (1.0 - hover);
end
